simulink model "Dual_Three_Leg_Inverter_DPWMA"  (R2023b)
settings: Solver=ode45  StartTime=0.0  StopTime=0.5  RelTol=1e-3  EnableMultiTasking=on
libraries: spsSeriesRLCBranchLib x12, spsCurrentMeasurementLib x7, spsRMSLib x3, spsVoltageMeasurementLib x3, simulink x2, spsMeanLib x2, spsTHDLib x2, spsUniversalBridgeLib x2, spsDCVoltageSourceLib x1, spspowerguiLib x1
settings Model: SimulationMode=accelerator  Creator=Administrator  LastModifiedBy=Qu
settings SolverCC: AlgebraicLoopSolver=TrustRegion
settings DataIOCC: LimitDataPoints=on  SaveFormat=Array  SignalLoggingSaveFormat=ModelDataLogs  ReturnWorkspaceOutputs=off
settings OptimizationCC: ExpressionDepthLimit=2147483647  LifeSpan=inf
settings DebuggingCC: UnderspecifiedInitializationDetection=Classic  MergeDetectMultiDrivingBlocksExec=none  SolverPrmCheckMsg=warning  FcnCallInpInsideContextMsg=warning  UnconnectedInputMsg=warning  UnconnectedOutputMsg=warning  UnconnectedLineMsg=warning  StateNameClashWarn=warning  SFUnexpectedBacktrackingDiag=warning  SFNoUnconditionalDefaultTransitionDiag=warning  SFExecutionAtInitializationDiag=none  ArithmeticOperatorsInVariantConditions=warning
settings HardwareCC: ProdBitPerPointer=32  ProdBitPerSizeT=32  ProdBitPerPtrDiffT=32  ProdLargestAtomicFloat=None  ProdIntDivRoundTo=Undefined  ProdEndianess=Unspecified  ProdWordSize=32  ProdHWDeviceType=32-bit Generic
settings ModelReferenceCC: EnableRefExpFcnMdlSchedulingChecks=on  PropagateSignalLabelsOutOfModel=off
settings SFSimCC: SimUseLocalCustomCode=off  CustomCodeUndefinedFunction=UseInterfaceOnly
settings RTWCC: RTWUseLocalCustomCode=off
settings CodeAppCC: StateflowObjectComments=on
settings GRTTargetCC: TargetLangStandard=C89/C90 (ANSI)  CombineOutputUpdateFcns=off  GRTInterface=on
settings ConfigComp: CovMetricSettings=dw  CovSaveCumulativeToWorkspaceVar=on  CovSaveSingleToWorkspaceVar=on  CovExternalEMLEnable=off
settings SimscapeCC: SimscapeNormalizeSystem=off

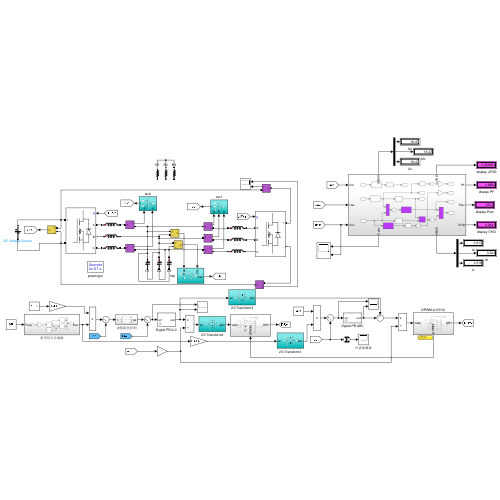
[thumbnail: Simulink's stored preview of the top-level diagram]
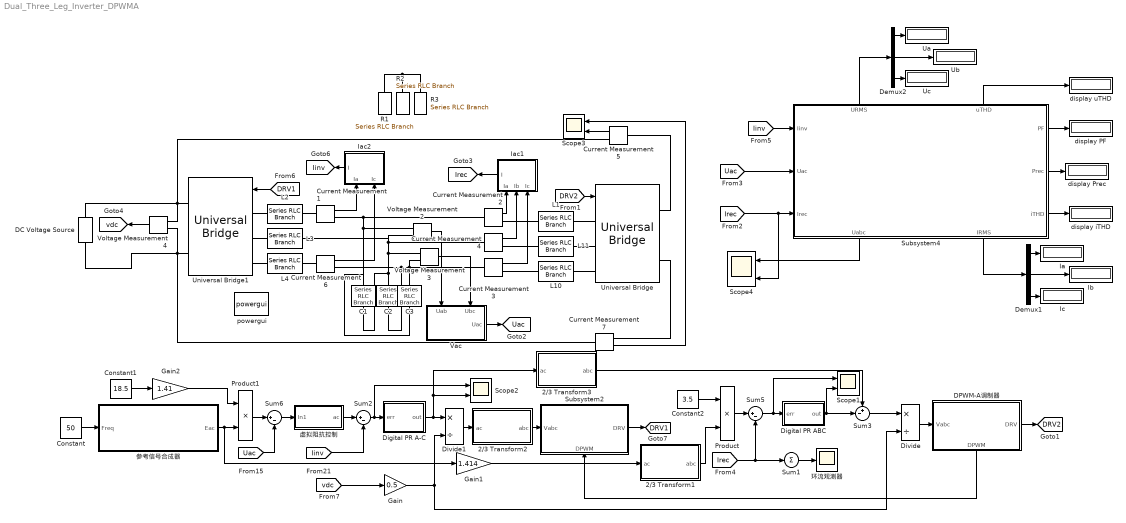
== system Dual_Three_Leg_Inverter_DPWMA ==
  2/3 Transform1 : Subsystem
      settings: PortSchema="{\"entries\":[{\"content\":{\"sides\":[{\"content\":{},\"type\":\"ConnectorPlacement.EquallySpacedRectSide\",\"uuid\":\"58c40194-9a95-4e39-952e-f878bde7484e\"},{\"content\":{\"side\":\"RIGHT\"},\"type\":\"ConnectorPlacement.EquallySpacedRectSide\",\"uuid\":\"f51692e8-3ff2-4d72-808d-3667196a4526\"},{\"content\":{\"connectorIds\":[\"In1\"],\"side\":\"TOP\"},\"type\":\"ConnectorPlacement.EquallySpacedRectSide\",\"uuid\":\"0aab136b-5da5-45c4-8998-999ebe8b7f2f\"},{\"content\":{\"connectorIds\":[\"Out1\"],\"side\":\"BOTTOM\"},\"type\":\"ConnectorPlacement.EquallySpacedRectSide\",\"uuid\":\"32f5f4a5-4ebb-496b-828d-b973bd46b44e\"}]},\"type\":\"ConnectorPlacement.EquallySpacedConnector\",\"uuid\":\"3ef81af7-d426-47fb-88e3-e33e58eebb83\"}],\"packageUris\":[\"http://schema.mathworks.com/mf0/Connector/R2020b\"],\"version\":\"1.0\"}"
  2/3 Transform2 : Subsystem
      settings: PortSchema="{\"entries\":[{\"content\":{\"sides\":[{\"content\":{},\"type\":\"ConnectorPlacement.EquallySpacedRectSide\",\"uuid\":\"58c40194-9a95-4e39-952e-f878bde7484e\"},{\"content\":{\"side\":\"RIGHT\"},\"type\":\"ConnectorPlacement.EquallySpacedRectSide\",\"uuid\":\"f51692e8-3ff2-4d72-808d-3667196a4526\"},{\"content\":{\"connectorIds\":[\"In1\"],\"side\":\"TOP\"},\"type\":\"ConnectorPlacement.EquallySpacedRectSide\",\"uuid\":\"0aab136b-5da5-45c4-8998-999ebe8b7f2f\"},{\"content\":{\"connectorIds\":[\"Out1\"],\"side\":\"BOTTOM\"},\"type\":\"ConnectorPlacement.EquallySpacedRectSide\",\"uuid\":\"32f5f4a5-4ebb-496b-828d-b973bd46b44e\"}]},\"type\":\"ConnectorPlacement.EquallySpacedConnector\",\"uuid\":\"3ef81af7-d426-47fb-88e3-e33e58eebb83\"}],\"packageUris\":[\"http://schema.mathworks.com/mf0/Connector/R2020b\"],\"version\":\"1.0\"}"
  2/3 Transform3 : Subsystem
      settings: PortSchema="{\"entries\":[{\"content\":{\"sides\":[{\"content\":{},\"type\":\"ConnectorPlacement.EquallySpacedRectSide\",\"uuid\":\"58c40194-9a95-4e39-952e-f878bde7484e\"},{\"content\":{\"side\":\"RIGHT\"},\"type\":\"ConnectorPlacement.EquallySpacedRectSide\",\"uuid\":\"f51692e8-3ff2-4d72-808d-3667196a4526\"},{\"content\":{\"connectorIds\":[\"In1\"],\"side\":\"TOP\"},\"type\":\"ConnectorPlacement.EquallySpacedRectSide\",\"uuid\":\"0aab136b-5da5-45c4-8998-999ebe8b7f2f\"},{\"content\":{\"connectorIds\":[\"Out1\"],\"side\":\"BOTTOM\"},\"type\":\"ConnectorPlacement.EquallySpacedRectSide\",\"uuid\":\"32f5f4a5-4ebb-496b-828d-b973bd46b44e\"}]},\"type\":\"ConnectorPlacement.EquallySpacedConnector\",\"uuid\":\"3ef81af7-d426-47fb-88e3-e33e58eebb83\"}],\"packageUris\":[\"http://schema.mathworks.com/mf0/Connector/R2020b\"],\"version\":\"1.0\"}"
  C1 : spsSeriesRLCBranchLib/Series RLC Branch  LConnTagsString=__new0  RConnTagsString=__new0  BranchType=C  Resistance=100  Inductance=1e-3  SetiL0=off  InitialCurrent=0  Capacitance=8e-6  Setx0=off  InitialVoltage=56  Measurements=None
  C2 : spsSeriesRLCBranchLib/Series RLC Branch  LConnTagsString=__new0  RConnTagsString=__new0  BranchType=C  Resistance=100  Inductance=1e-3  SetiL0=off  InitialCurrent=0  Capacitance=8e-6  Setx0=off  InitialVoltage=56  Measurements=None
  C3 : spsSeriesRLCBranchLib/Series RLC Branch  LConnTagsString=__new0  RConnTagsString=__new0  BranchType=C  Resistance=100  Inductance=1e-3  SetiL0=off  InitialCurrent=0  Capacitance=8e-6  Setx0=off  InitialVoltage=56  Measurements=None
  Constant : Constant  Value=50
  Constant1 : Constant  Value=18.5
  Constant2 : Constant  Value=3.5
  Current Measurement{1..7} (7 alike) : spsCurrentMeasurementLib/Current Measurement  PhasorSimulation=off  OutputType=Complex  PSBequivalent=0
  DC Voltage Source : spsDCVoltageSourceLib/DC Voltage Source  Amplitude=50  Measurements=None
  DPWM-A调制器 : Subsystem
      settings: PortSchema="{\"entries\":[{\"content\":{\"sides\":[{\"content\":{\"connectorIds\":[\"In1\"]},\"type\":\"ConnectorPlacement.EquallySpacedRectSide\",\"uuid\":\"1b921e88-89d9-40c8-80a6-19c9bba63005\"},{\"content\":{\"connectorIds\":[\"Out1\"],\"side\":\"RIGHT\"},\"type\":\"ConnectorPlacement.EquallySpacedRectSide\",\"uuid\":\"19f123f7-b197-44a6-b6a2-b5017f4a2a93\"},{\"content\":{\"side\":\"TOP\"},\"type\":\"ConnectorPlacement.EquallySpacedRectSide\",\"uuid\":\"1cf9155b-da68-48e1-b9a8-e44105d4bd88\"},{\"content\":{\"connectorIds\":[\"Out2\"],\"side\":\"BOTTOM\"},\"type\":\"ConnectorPlacement.EquallySpacedRectSide\",\"uuid\":\"2b44f05d-f684-4967-9c90-42e6d34a3f81\"}]},\"type\":\"ConnectorPlacement.EquallySpacedConnector\",\"uuid\":\"7b9a8e17-ffb5-4515-884d-b733a1796f36\"}],\"packageUris\":[\"http://schema.mathworks.com/mf0/Connector/R2020b\"],\"version\":\"1.0\"}"
  Demux1 : Demux  Outputs=3
  Demux2 : Demux  Outputs=3
  Digital PR A-C : Subsystem  mask{Kp=5, Kr=100, Wc=5, Ts=1/40000, Upper=80, Lower=-80}
      mask DialogControl ParameterGroupVar Prompt: 参数
  Digital PR ABC : Subsystem  mask{Kp=5, Kr=100, Wc=5, Ts=1/40000, Upper=80, Lower=-80}
      mask DialogControl ParameterGroupVar Prompt: 参数
  Divide : Product  Inputs=*/
  Divide1 : Product  Inputs=*/
  Gain : Gain  Gain=0.5
  Gain1 : Gain  Gain=1.414
  Gain2 : Gain  Gain=1.41
  Ia : Display
  Iac1 : Subsystem
      settings: PortSchema="{\"entries\":[{\"content\":{\"sides\":[{\"content\":{\"connectorIds\":[\"In1\",\"In2\",\"In3\"]},\"type\":\"ConnectorPlacement.EquallySpacedRectSide\",\"uuid\":\"58c40194-9a95-4e39-952e-f878bde7484e\"},{\"content\":{\"side\":\"RIGHT\"},\"type\":\"ConnectorPlacement.EquallySpacedRectSide\",\"uuid\":\"f51692e8-3ff2-4d72-808d-3667196a4526\"},{\"content\":{\"side\":\"TOP\"},\"type\":\"ConnectorPlacement.EquallySpacedRectSide\",\"uuid\":\"0aab136b-5da5-45c4-8998-999ebe8b7f2f\"},{\"content\":{\"connectorIds\":[\"Out1\"],\"side\":\"BOTTOM\"},\"type\":\"ConnectorPlacement.EquallySpacedRectSide\",\"uuid\":\"32f5f4a5-4ebb-496b-828d-b973bd46b44e\"}]},\"type\":\"ConnectorPlacement.EquallySpacedConnector\",\"uuid\":\"3ef81af7-d426-47fb-88e3-e33e58eebb83\"}],\"packageUris\":[\"http://schema.mathworks.com/mf0/Connector/R2020b\"],\"version\":\"1.0\"}"
  Iac2 : Subsystem
      settings: PortSchema="{\"entries\":[{\"content\":{\"sides\":[{\"content\":{\"connectorIds\":[\"In1\",\"In2\"]},\"type\":\"ConnectorPlacement.EquallySpacedRectSide\",\"uuid\":\"58c40194-9a95-4e39-952e-f878bde7484e\"},{\"content\":{\"side\":\"RIGHT\"},\"type\":\"ConnectorPlacement.EquallySpacedRectSide\",\"uuid\":\"f51692e8-3ff2-4d72-808d-3667196a4526\"},{\"content\":{\"side\":\"TOP\"},\"type\":\"ConnectorPlacement.EquallySpacedRectSide\",\"uuid\":\"0aab136b-5da5-45c4-8998-999ebe8b7f2f\"},{\"content\":{\"connectorIds\":[\"Out1\"],\"side\":\"BOTTOM\"},\"type\":\"ConnectorPlacement.EquallySpacedRectSide\",\"uuid\":\"32f5f4a5-4ebb-496b-828d-b973bd46b44e\"}]},\"type\":\"ConnectorPlacement.EquallySpacedConnector\",\"uuid\":\"3ef81af7-d426-47fb-88e3-e33e58eebb83\"}],\"packageUris\":[\"http://schema.mathworks.com/mf0/Connector/R2020b\"],\"version\":\"1.0\"}"
  Ib : Display
  Ic : Display
  L1 : spsSeriesRLCBranchLib/Series RLC Branch  LConnTagsString=__new0  RConnTagsString=__new0  BranchType=L  Resistance=1  Inductance=3e-4  SetiL0=off  InitialCurrent=0  Capacitance=2e-3  Setx0=off  InitialVoltage=0  Measurements=None
  L10 : spsSeriesRLCBranchLib/Series RLC Branch  LConnTagsString=__new0  RConnTagsString=__new0  BranchType=L  Resistance=1  Inductance=3e-4  SetiL0=off  InitialCurrent=0  Capacitance=2e-3  Setx0=off  InitialVoltage=0  Measurements=None
  L11 : spsSeriesRLCBranchLib/Series RLC Branch  LConnTagsString=__new0  RConnTagsString=__new0  BranchType=L  Resistance=1  Inductance=3e-4  SetiL0=off  InitialCurrent=0  Capacitance=2e-3  Setx0=off  InitialVoltage=0  Measurements=None
  L2 : spsSeriesRLCBranchLib/Series RLC Branch  LConnTagsString=__new0  RConnTagsString=__new0  BranchType=L  Resistance=0.1  Inductance=3e-4  SetiL0=off  InitialCurrent=0  Capacitance=2e-3  Setx0=off  InitialVoltage=0  Measurements=None
  L3 : spsSeriesRLCBranchLib/Series RLC Branch  LConnTagsString=__new0  RConnTagsString=__new0  BranchType=L  Resistance=0.1  Inductance=3e-4  SetiL0=off  InitialCurrent=0  Capacitance=2e-3  Setx0=off  InitialVoltage=0  Measurements=None
  L4 : spsSeriesRLCBranchLib/Series RLC Branch  LConnTagsString=__new0  RConnTagsString=__new0  BranchType=L  Resistance=0.1  Inductance=3e-4  SetiL0=off  InitialCurrent=0  Capacitance=2e-3  Setx0=off  InitialVoltage=0  Measurements=None
  Product : Product
  Product1 : Product
  R1 : spsSeriesRLCBranchLib/Series RLC Branch  LConnTagsString=__new0  RConnTagsString=__new0  BranchType=R  Resistance=10  Inductance=1e-3  SetiL0=off  InitialCurrent=0  Capacitance=2e-3  Setx0=on  InitialVoltage=540  Measurements=None
  R2 : spsSeriesRLCBranchLib/Series RLC Branch  LConnTagsString=__new0  RConnTagsString=__new0  BranchType=R  Resistance=10  Inductance=1e-3  SetiL0=off  InitialCurrent=0  Capacitance=2e-3  Setx0=on  InitialVoltage=540  Measurements=None
  R3 : spsSeriesRLCBranchLib/Series RLC Branch  LConnTagsString=__new0  RConnTagsString=__new0  BranchType=R  Resistance=10  Inductance=1e-3  SetiL0=off  InitialCurrent=0  Capacitance=2e-3  Setx0=on  InitialVoltage=540  Measurements=None
  Scope{1..4} (4 alike) : Scope  NumInputPorts=2
  Subsystem2 : Subsystem
      settings: PortSchema="{\"entries\":[{\"content\":{\"sides\":[{\"content\":{\"connectorIds\":[\"In1\"]},\"type\":\"ConnectorPlacement.EquallySpacedRectSide\",\"uuid\":\"de8b90f0-7b55-4abd-a179-300fa705da97\"},{\"content\":{\"connectorIds\":[\"Out1\"],\"side\":\"RIGHT\"},\"type\":\"ConnectorPlacement.EquallySpacedRectSide\",\"uuid\":\"0792874a-d250-4054-8a74-d5389a9b2639\"},{\"content\":{\"side\":\"TOP\"},\"type\":\"ConnectorPlacement.EquallySpacedRectSide\",\"uuid\":\"613a9447-7ac5-4140-b452-30bec5459d5a\"},{\"content\":{\"connectorIds\":[\"In2\"],\"side\":\"BOTTOM\"},\"type\":\"ConnectorPlacement.EquallySpacedRectSide\",\"uuid\":\"fd3fd695-8830-4e72-9238-e853f444166a\"}]},\"type\":\"ConnectorPlacement.EquallySpacedConnector\",\"uuid\":\"d7512945-9f99-49d8-b46f-637000ed2988\"}],\"packageUris\":[\"http://schema.mathworks.com/mf0/Connector/R2020b\"],\"version\":\"1.0\"}"
  Subsystem4 : Subsystem
      settings: PortSchema="{\"entries\":[{\"content\":{\"sides\":[{\"content\":{\"connectorIds\":[\"In1\",\"In2\",\"In3\"]},\"type\":\"ConnectorPlacement.EquallySpacedRectSide\",\"uuid\":\"8f3b7bf1-7c44-4492-a357-aa6e3e6d66a4\"},{\"content\":{\"connectorIds\":[\"Out1\",\"Out2\",\"Out3\"],\"side\":\"RIGHT\"},\"type\":\"ConnectorPlacement.EquallySpacedRectSide\",\"uuid\":\"7ae784cf-6bcf-4684-9c07-1770fc60c8a0\"},{\"content\":{\"connectorIds\":[\"Out6\",\"Out7\"],\"side\":\"TOP\"},\"type\":\"ConnectorPlacement.EquallySpacedRectSide\",\"uuid\":\"0e016931-6232-4ad6-afe9-572a0571336f\"},{\"content\":{\"connectorIds\":[\"Out4\",\"Out5\"],\"side\":\"BOTTOM\"},\"type\":\"ConnectorPlacement.EquallySpacedRectSide\",\"uuid\":\"ef67c6ee-ba81-4705-af34-81581e7e9907\"}]},\"type\":\"ConnectorPlacement.EquallySpacedConnector\",\"uuid\":\"922af512-c0ff-443f-816c-194775a78dc8\"}],\"packageUris\":[\"http://schema.mathworks.com/mf0/Connector/R2020b\"],\"version\":\"1.0\"}"
  Sum1 : Sum  Inputs=+
  Sum2 : Sum  Inputs=|+-
  Sum3 : Sum  Inputs=+-|
  Sum5 : Sum  Inputs=|+-
  Sum6 : Sum  Inputs=|+-
  Ua : Display
  Ub : Display
  Uc : Display
  Universal Bridge : spsUniversalBridgeLib/Universal Bridge  Arms=3  SnubberResistance=1e5  SnubberCapacitance=inf  Device=MOSFET / Diodes  Ron=1e-3  Lon=0  ForwardVoltages="[  0  0  ]"  ForwardVoltage=0  GTOparameters=[ 10e-6 , 20e-6 ]  IGBTparameters=[ 1e-6 , 2e-6 ]  Measurements=None  Measurements_2=None  converterType=Rectifier
  Universal Bridge1 : spsUniversalBridgeLib/Universal Bridge  Arms=3  SnubberResistance=1e5  SnubberCapacitance=inf  Device=MOSFET / Diodes  Ron=1e-3  Lon=0  ForwardVoltages="[  0  0  ]"  ForwardVoltage=0  GTOparameters=[ 10e-6 , 20e-6 ]  IGBTparameters=[ 1e-6 , 2e-6 ]  Measurements=None  Measurements_2=None  converterType=Rectifier
  Vac : Subsystem
      settings: PortSchema="{\"entries\":[{\"content\":{\"sides\":[{\"content\":{\"connectorIds\":[\"In1\",\"In2\"]},\"type\":\"ConnectorPlacement.EquallySpacedRectSide\",\"uuid\":\"58c40194-9a95-4e39-952e-f878bde7484e\"},{\"content\":{\"connectorIds\":[],\"side\":\"RIGHT\"},\"type\":\"ConnectorPlacement.EquallySpacedRectSide\",\"uuid\":\"f51692e8-3ff2-4d72-808d-3667196a4526\"},{\"content\":{\"connectorIds\":[],\"side\":\"TOP\"},\"type\":\"ConnectorPlacement.EquallySpacedRectSide\",\"uuid\":\"0aab136b-5da5-45c4-8998-999ebe8b7f2f\"},{\"content\":{\"connectorIds\":[\"Out1\"],\"side\":\"BOTTOM\"},\"type\":\"ConnectorPlacement.EquallySpacedRectSide\",\"uuid\":\"185ce796-68e2-4136-8080-97dc86d2ba54\"}]},\"type\":\"ConnectorPlacement.EquallySpacedConnector\",\"uuid\":\"3ef81af7-d426-47fb-88e3-e33e58eebb83\"}],\"packageUris\":[\"http://schema.mathworks.com/mf0/Connector/R2020b\"],\"version\":\"1.0\"}"
  Voltage Measurement2 : spsVoltageMeasurementLib/Voltage Measurement  PhasorSimulation=off  OutputType=Complex  PSBequivalent=0
  Voltage Measurement3 : spsVoltageMeasurementLib/Voltage Measurement  PhasorSimulation=off  OutputType=Complex  PSBequivalent=0
  Voltage Measurement4 : spsVoltageMeasurementLib/Voltage Measurement  PhasorSimulation=off  OutputType=Complex  PSBequivalent=0
  display PF : Display
  display Prec : Display
  display iTHD : Display
  display uTHD : Display
  powergui : spspowerguiLib/powergui  Priority=1  SimulationMode=Discrete  SampleTime=2e-7  frequency=60  Iterations=50  frequencyindice=0  Pbase=100e6  ErrMax=1e-4  UnitsV=kV  UnitsW=MW  buscounter=0  FunctionMessages=off  echomessages=off  EnableUseOfTLC=off  CurrentSourceSwitches=off  DisableSnubberDevices=off  DisableRonSwitches=off  DisableVfSwitches=off  DisplayEquations=off  AutomaticDiscreteSolvers=off  SolverType=Tustin  Interpol=off  ExternalGateDelay=off  methode=off  Ts=0  x0status=blocks  SPID=off  SwTol=0  HookPort=off  NonlinearTolerance=1e-4  nMaxIteration=100  ContinueOnMaxIteration=off  RestoreLinks=warning  ResistiveCurrentMeasurement=off  Frange=[0:2:500]  Ylog=off  Xlog=on  ShowGrid=off  save=off  variable=ZData  structure=0  ZoomFFT=off  StartTime=0.0  cycles=1  DisplayStyle=1  fundamental=60  FreqAxis=off  MaxFrequency=1000  frequencyindicesteady=1  RmsSteady=1  display=off
  参考信号合成器 : Subsystem
  环流观测器 : Scope
  虚拟阻抗控制 : Subsystem
  tag scope: DRV1=global, DRV2=global, Iinv=global, Irec=global, Uac=global, vdc=global
  wires:
  [DRV2] -> Universal Bridge/1
  [Irec] -> Sum1/1, Sum5/2
  Sum5/1 -> Scope1/1, Digital PR ABC/1(err)
  Digital PR ABC/1(out) -> Scope1/2, Sum3/2
  Voltage Measurement2/1 -> Vac/1(Uab)
  Voltage Measurement3/1 -> Vac/2(Ubc)
  Vac/1(Uac) -> [Uac]
  Subsystem4/1(PF) -> display PF/1
  Subsystem4/3(iTHD) -> display iTHD/1
  [Iinv] -> Subsystem4/1(Iinv)
  Product/1 -> Sum5/1
  Sum3/1 -> Divide/1
  [Irec] -> Scope4/2, Subsystem4/3(Irec)
  [Uac] -> Subsystem4/2(Uac)
  Current Measurement1/1 -> Iac2/2(Ia)
  Iac2/1(I) -> [Iinv]
  Constant/1 -> 参考信号合成器/1(Freq)
  Sum6/1 -> 虚拟阻抗控制/1(In1)
  [Iinv] -> Sum2/2
  [Uac] -> Sum6/2
  参考信号合成器/1(Eac) -> Gain1/1, Product1/2
  Gain2/1 -> Product1/1
  Constant1/1 -> Gain2/1
  Product1/1 -> Sum6/1
  [DRV1] -> Universal Bridge1/1
  Current Measurement2/1 -> Iac1/3(Ia)
  Iac1/1(I) -> [Irec]
  Current Measurement3/1 -> Iac1/1(Ic)
  Current Measurement4/1 -> Iac1/2(Ib)
  Subsystem2/1(DRV) -> [DRV1]
  Voltage Measurement4/1 -> [vdc]
  Current Measurement5/1 -> Scope3/2
  Current Measurement7/1 -> Scope3/1
  Constant2/1 -> Product/1
  Current Measurement6/1 -> Iac2/1(Ic)
  Sum2/1 -> Scope2/1, Digital PR A-C/1(err)
  2/3 Transform1/1(abc) -> Product/2
  虚拟阻抗控制/1(ac) -> Sum2/1
  Divide1/1 -> 2/3 Transform2/1(ac)
  DPWM-A调制器/1(DRV) -> [DRV2]
  [vdc] -> Gain/1
  Gain/1 -> Divide/2, Divide1/2
  Divide/1 -> DPWM-A调制器/1(Vabc)
  Sum1/1 -> 环流观测器/1
  2/3 Transform2/1(abc) -> Subsystem2/1(Vabc)
  2/3 Transform3/1(abc) -> Sum3/1
  Digital PR A-C/1(out) -> Divide1/1, 2/3 Transform3/1(ac), Scope2/2
  Demux2/3 -> Uc/1
  Demux2/1 -> Ua/1
  Demux2/2 -> Ub/1
  Subsystem4/6(URMS) -> Demux2/1
  Subsystem4/2(Prec) -> display Prec/1
  Subsystem4/7(uTHD) -> display uTHD/1
  Subsystem4/4(Uabc) -> Scope4/1
  Subsystem4/5(IRMS) -> Demux1/1
  Demux1/2 -> Ib/1
  Demux1/1 -> Ia/1
  Demux1/3 -> Ic/1
  Gain1/1 -> 2/3 Transform1/1(ac)
  DPWM-A调制器/2(DPWM) -> Subsystem2/2(DPWM)
  connections:
  L1/RConn1 -- Universal Bridge/LConn1
  L11/RConn1 -- Universal Bridge/LConn2
  L2/RConn1 -- Current Measurement1/LConn1
  Current Measurement1/RConn1 -- Current Measurement2/LConn1 -- C3/RConn1 -- C1/LConn1 -- Voltage Measurement2/LConn1
  Current Measurement2/RConn1 -- L1/LConn1
  L10/RConn1 -- Universal Bridge/LConn3
  Universal Bridge1/LConn1 -- L2/LConn1
  L3/LConn1 -- Universal Bridge1/LConn2
  L4/LConn1 -- Universal Bridge1/LConn3
  L4/RConn1 -- Current Measurement6/LConn1
  C2/LConn1 -- Current Measurement4/LConn1 -- Voltage Measurement2/LConn2 -- L3/RConn1 -- Voltage Measurement3/LConn1 -- C1/RConn1
  C3/LConn1 -- Current Measurement3/LConn1 -- Voltage Measurement3/LConn2 -- Current Measurement6/RConn1 -- C2/RConn1
  Current Measurement3/RConn1 -- L10/LConn1
  Current Measurement4/RConn1 -- L11/LConn1
  Voltage Measurement4/LConn1 -- Universal Bridge1/RConn1 -- Current Measurement5/RConn1 -- DC Voltage Source/RConn1
  Voltage Measurement4/LConn2 -- Current Measurement7/LConn1 -- DC Voltage Source/LConn1 -- Universal Bridge1/RConn2
  Current Measurement5/LConn1 -- Universal Bridge/RConn1
  Current Measurement7/RConn1 -- Universal Bridge/RConn2
  R1/RConn1 -- R3/RConn1 -- R2/RConn1

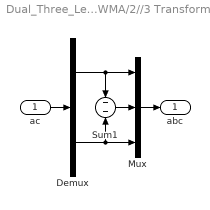
== system Dual_Three_Leg_Inverter_DPWMA/2//3 Transform1 ==
  ac : Inport
  Demux : Demux  Outputs=2
  Mux : Mux  Inputs=3
  Sum1 : Sum  Inputs=-|-
  abc : Outport
  wires:
  Demux/2 -> Mux/3, Sum1/2
  ac/1 -> Demux/1
  Demux/1 -> Mux/1, Sum1/1
  Mux/1 -> abc/1
  Sum1/1 -> Mux/2

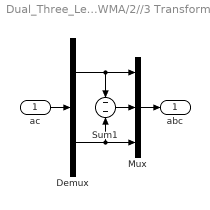
== system Dual_Three_Leg_Inverter_DPWMA/2//3 Transform2 ==
  ac : Inport
  Demux : Demux  Outputs=2
  Mux : Mux  Inputs=3
  Sum1 : Sum  Inputs=-|-
  abc : Outport
  wires:
  Sum1/1 -> Mux/2
  Mux/1 -> abc/1
  Demux/1 -> Sum1/1, Mux/1
  ac/1 -> Demux/1
  Demux/2 -> Sum1/2, Mux/3

== system Dual_Three_Leg_Inverter_DPWMA/2//3 Transform3 ==
  ac : Inport
  Demux : Demux  Outputs=2
  Mux : Mux  Inputs=3
  Sum1 : Sum  Inputs=-|-
  abc : Outport
  wires:
  Sum1/1 -> Mux/2
  Mux/1 -> abc/1
  Demux/1 -> Sum1/1, Mux/1
  ac/1 -> Demux/1
  Demux/2 -> Sum1/2, Mux/3

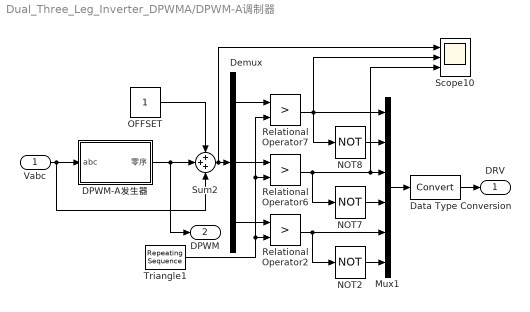
== system Dual_Three_Leg_Inverter_DPWMA/DPWM-A调制器 ==
  Vabc : Inport
  DPWM-A发生器 : Subsystem
  Data Type Conversion : DataTypeConversion  SaturateOnIntegerOverflow=off  RndMeth=Floor
  Demux : Demux  Outputs=3
  Mux1 : Mux  Inputs=6
  NOT2 : Logic  Operator=NOT  IconShape=distinctive  AllPortsSameDT=off  OutDataTypeStr=boolean
  NOT7 : Logic  Operator=NOT  IconShape=distinctive  AllPortsSameDT=off  OutDataTypeStr=boolean
  NOT8 : Logic  Operator=NOT  IconShape=distinctive  AllPortsSameDT=off  OutDataTypeStr=boolean
  OFFSET : Constant
  Relational Operator2 : RelationalOperator  Operator=>  OutDataTypeStr=boolean  InputSameDT=off
  Relational Operator6 : RelationalOperator  Operator=>  OutDataTypeStr=boolean  InputSameDT=off
  Relational Operator7 : RelationalOperator  Operator=>  OutDataTypeStr=boolean  InputSameDT=off
  Scope10 : Scope  NumInputPorts=3
  Sum2 : Sum  Inputs=+++
  Triangle1 : simulink/Sources/Repeating Sequence  rep_seq_t=[0 1/20000/2 1/20000]  rep_seq_y=[0 2 0]
  DRV : Outport
  DPWM : Outport  Port=2
  wires:
  Vabc/1 -> DPWM-A发生器/1(abc), Sum2/3
  Relational Operator6/1 -> Scope10/3, Mux1/3, NOT7/1
  NOT7/1 -> Mux1/4
  Relational Operator7/1 -> NOT8/1, Scope10/2, Mux1/1
  Triangle1/1 -> Relational Operator2/2, Relational Operator7/2, Relational Operator6/2
  NOT8/1 -> Mux1/2
  Relational Operator2/1 -> Mux1/5, NOT2/1
  NOT2/1 -> Mux1/6
  Demux/1 -> Relational Operator7/1
  Demux/2 -> Relational Operator6/1
  Demux/3 -> Relational Operator2/1
  Sum2/1 -> Scope10/1, Demux/1
  Mux1/1 -> Data Type Conversion/1
  Data Type Conversion/1 -> DRV/1
  OFFSET/1 -> Sum2/1
  DPWM-A发生器/1(零序) -> DPWM/1, Sum2/2

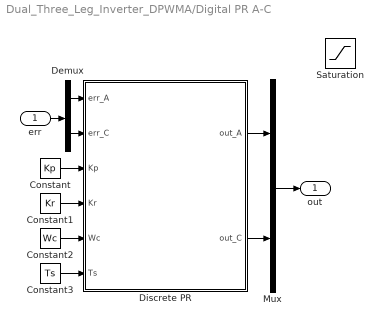
== system Dual_Three_Leg_Inverter_DPWMA/Digital PR A-C ==
  err : Inport
  Constant : Constant  Value=Kp
  Constant1 : Constant  Value=Kr
  Constant2 : Constant  Value=Wc
  Constant3 : Constant  Value=Ts
  Demux : Demux  Outputs=2
  Discrete PR : MATLAB Function  TreatAsAtomicUnit=on
  Mux : Mux  Inputs=2
  Saturation : Saturate  UpperLimit=Upper  LowerLimit=Lower
  out : Outport
  wires:
  Constant1/1 -> Discrete PR/4(Kr)
  Constant3/1 -> Discrete PR/6(Ts)
  Constant/1 -> Discrete PR/3(Kp)
  Constant2/1 -> Discrete PR/5(Wc)
  Demux/1 -> Discrete PR/1(err_A)
  err/1 -> Demux/1
  Demux/2 -> Discrete PR/2(err_C)
  Discrete PR/1(out_A) -> Mux/1
  Discrete PR/2(out_C) -> Mux/2
  Mux/1 -> out/1

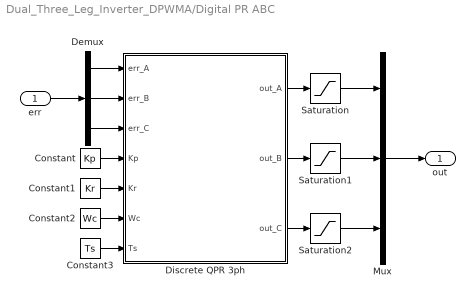
== system Dual_Three_Leg_Inverter_DPWMA/Digital PR ABC ==
  err : Inport
  Constant : Constant  Value=Kp
  Constant1 : Constant  Value=Kr
  Constant2 : Constant  Value=Wc
  Constant3 : Constant  Value=Ts
  Demux : Demux  Outputs=3
  Discrete QPR 3ph : MATLAB Function  TreatAsAtomicUnit=on
  Mux : Mux  Inputs=3
  Saturation : Saturate  UpperLimit=Upper  LowerLimit=Lower
  Saturation1 : Saturate  UpperLimit=Upper  LowerLimit=Lower
  Saturation2 : Saturate  UpperLimit=Upper  LowerLimit=Lower
  out : Outport
  wires:
  Discrete QPR 3ph/1(out_A) -> Saturation/1
  Constant1/1 -> Discrete QPR 3ph/5(Kr)
  Constant3/1 -> Discrete QPR 3ph/7(Ts)
  Constant/1 -> Discrete QPR 3ph/4(Kp)
  Constant2/1 -> Discrete QPR 3ph/6(Wc)
  Discrete QPR 3ph/2(out_B) -> Saturation1/1
  Discrete QPR 3ph/3(out_C) -> Saturation2/1
  Demux/2 -> Discrete QPR 3ph/2(err_B)
  Demux/3 -> Discrete QPR 3ph/3(err_C)
  Demux/1 -> Discrete QPR 3ph/1(err_A)
  err/1 -> Demux/1
  Saturation2/1 -> Mux/3
  Saturation1/1 -> Mux/2
  Saturation/1 -> Mux/1
  Mux/1 -> out/1

== system Dual_Three_Leg_Inverter_DPWMA/Iac1 ==
  Ic : Inport
  Ib : Inport  Port=2
  Ia : Inport  Port=3
  Mux : Mux  Inputs=3
  I : Outport
  wires:
  Ia/1 -> Mux/1
  Ib/1 -> Mux/2
  Mux/1 -> I/1
  Ic/1 -> Mux/3

== system Dual_Three_Leg_Inverter_DPWMA/Iac2 ==
  Ic : Inport
  Ia : Inport  Port=2
  Mux : Mux  Inputs=2
  I : Outport
  wires:
  Mux/1 -> I/1
  Ia/1 -> Mux/1
  Ic/1 -> Mux/2

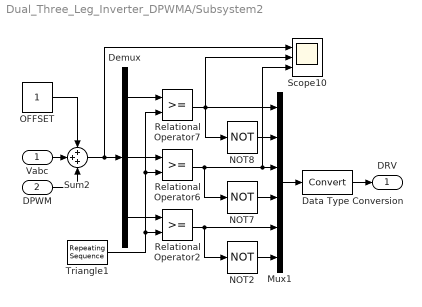
== system Dual_Three_Leg_Inverter_DPWMA/Subsystem2 ==
  Vabc : Inport
  DPWM : Inport  Port=2
  Data Type Conversion : DataTypeConversion  SaturateOnIntegerOverflow=off  RndMeth=Floor
  Demux : Demux  Outputs=3
  Mux1 : Mux  Inputs=6
  NOT2 : Logic  Operator=NOT  IconShape=distinctive  AllPortsSameDT=off  OutDataTypeStr=boolean
  NOT7 : Logic  Operator=NOT  IconShape=distinctive  AllPortsSameDT=off  OutDataTypeStr=boolean
  NOT8 : Logic  Operator=NOT  IconShape=distinctive  AllPortsSameDT=off  OutDataTypeStr=boolean
  OFFSET : Constant
  Relational Operator2 : RelationalOperator  OutDataTypeStr=boolean  InputSameDT=off
  Relational Operator6 : RelationalOperator  OutDataTypeStr=boolean  InputSameDT=off
  Relational Operator7 : RelationalOperator  OutDataTypeStr=boolean  InputSameDT=off
  Scope10 : Scope  NumInputPorts=3
  Sum2 : Sum  Inputs=+++
  Triangle1 : simulink/Sources/Repeating Sequence  rep_seq_t=[0 1/20000/2 1/20000]  rep_seq_y=[0 2 0]
  DRV : Outport
  wires:
  OFFSET/1 -> Sum2/1
  Data Type Conversion/1 -> DRV/1
  Mux1/1 -> Data Type Conversion/1
  Sum2/1 -> Scope10/1, Demux/1
  Demux/3 -> Relational Operator2/1
  Demux/2 -> Relational Operator6/1
  Demux/1 -> Relational Operator7/1
  NOT2/1 -> Mux1/6
  Relational Operator2/1 -> NOT2/1, Mux1/5
  NOT8/1 -> Mux1/2
  Relational Operator7/1 -> NOT8/1, Scope10/2, Mux1/1
  NOT7/1 -> Mux1/4
  Relational Operator6/1 -> NOT7/1, Scope10/3, Mux1/3
  DPWM/1 -> Sum2/3
  Vabc/1 -> Sum2/2
  Triangle1/1 -> Relational Operator7/2, Relational Operator6/2, Relational Operator2/2

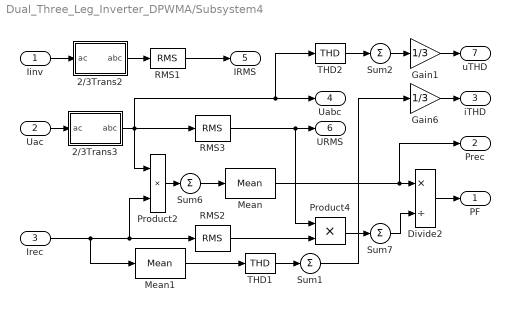
== system Dual_Three_Leg_Inverter_DPWMA/Subsystem4 ==
  Iinv : Inport
  Uac : Inport  Port=2
  Irec : Inport  Port=3
  2/3Trans2 : Subsystem
  2/3Trans3 : Subsystem
  Divide2 : Product  Inputs=*/
  Gain1 : Gain  Gain=1/3
  Gain6 : Gain  Gain=1/3
  Mean : spsMeanLib/Mean  Freq=100  Vinit=0  Ts=0
  Mean1 : spsMeanLib/Mean  Freq=5000  Vinit=0  Ts=0
  Product2 : Product
  Product4 : Product
  RMS1 : spsRMSLib/RMS  TrueRMS=on  Freq=50  RMSInit=0  Ts=0
  RMS2 : spsRMSLib/RMS  TrueRMS=on  Freq=50  RMSInit=0  Ts=0
  RMS3 : spsRMSLib/RMS  TrueRMS=on  Freq=50  RMSInit=0  Ts=0
  Sum{1..2,6..7} (4 alike) : Sum  Inputs=+
  THD1 : spsTHDLib/THD  Freq=50  Ts=0
  THD2 : spsTHDLib/THD  Freq=50  Ts=0
  PF : Outport
  Prec : Outport  Port=2
  iTHD : Outport  Port=3
  Uabc : Outport  Port=4
  IRMS : Outport  Port=5
  URMS : Outport  Port=6
  uTHD : Outport  Port=7
  wires:
  RMS1/1 -> IRMS/1
  2/3Trans2/1(abc) -> RMS1/1
  Iinv/1 -> 2/3Trans2/1(ac)
  Irec/1 -> Mean1/1, Product2/2, RMS2/1
  Product2/1 -> Sum6/1
  2/3Trans3/1(abc) -> Uabc/1, THD2/1, Product2/1, RMS3/1
  Uac/1 -> 2/3Trans3/1(ac)
  Product4/1 -> Sum7/1
  Sum7/1 -> Divide2/2
  RMS3/1 -> URMS/1, Product4/1
  THD1/1 -> Sum1/1
  RMS2/1 -> Product4/2
  Divide2/1 -> PF/1
  Sum6/1 -> Mean/1
  Gain6/1 -> iTHD/1
  Mean/1 -> Prec/1, Divide2/1
  Sum1/1 -> Gain6/1
  THD2/1 -> Sum2/1
  Sum2/1 -> Gain1/1
  Gain1/1 -> uTHD/1
  Mean1/1 -> THD1/1

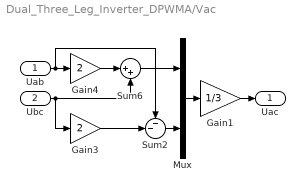
== system Dual_Three_Leg_Inverter_DPWMA/Vac ==
  Uab : Inport
  Ubc : Inport  Port=2
  Gain1 : Gain  Gain=1/3
  Gain3 : Gain  Gain=2
  Gain4 : Gain  Gain=2
  Mux : Mux  Inputs=2
  Sum2 : Sum  Inputs=--|
  Sum6 : Sum  Inputs=|++
  Uac : Outport
  wires:
  Uab/1 -> Sum2/1, Gain4/1
  Gain4/1 -> Sum6/1
  Ubc/1 -> Gain3/1, Sum6/2
  Gain3/1 -> Sum2/2
  Mux/1 -> Gain1/1
  Gain1/1 -> Uac/1
  Sum6/1 -> Mux/1
  Sum2/1 -> Mux/2

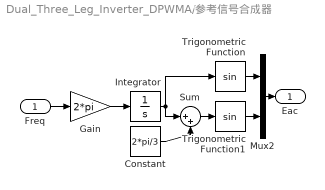
== system Dual_Three_Leg_Inverter_DPWMA/参考信号合成器 ==
  Freq : Inport
  Constant : Constant  Value=2*pi/3
  Gain : Gain  Gain=2*pi
  Integrator : Integrator  WrapState=on  WrappedStateUpperValue=2*pi  WrappedStateLowerValue=0
  Mux2 : Mux  Inputs=2
  Sum : Sum  Inputs=|++
  Trigonometric Function : Trigonometry
  Trigonometric Function1 : Trigonometry
  Eac : Outport
  wires:
  Gain/1 -> Integrator/1
  Freq/1 -> Gain/1
  Integrator/1 -> Trigonometric Function/1, Sum/1
  Constant/1 -> Sum/2
  Sum/1 -> Trigonometric Function1/1
  Trigonometric Function/1 -> Mux2/1
  Mux2/1 -> Eac/1
  Trigonometric Function1/1 -> Mux2/2

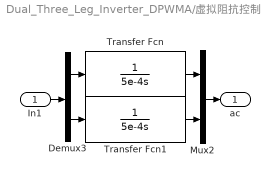
== system Dual_Three_Leg_Inverter_DPWMA/虚拟阻抗控制 ==
  In1 : Inport
  Demux3 : Demux  Outputs=2
  Mux2 : Mux  Inputs=2
  Transfer Fcn : TransferFcn  Denominator=[5e-4 0]
  Transfer Fcn1 : TransferFcn  Denominator=[5e-4 0]
  ac : Outport
  wires:
  Transfer Fcn/1 -> Mux2/1
  Mux2/1 -> ac/1
  Demux3/1 -> Transfer Fcn/1
  In1/1 -> Demux3/1
  Demux3/2 -> Transfer Fcn1/1
  Transfer Fcn1/1 -> Mux2/2

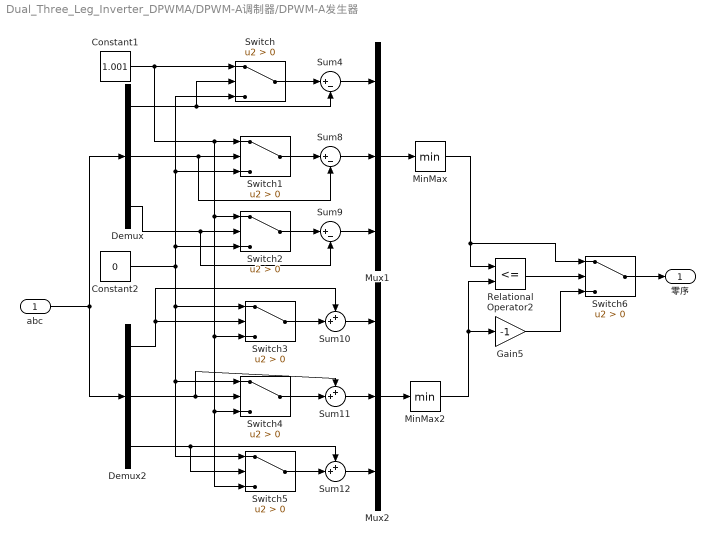
== system Dual_Three_Leg_Inverter_DPWMA/DPWM-A调制器/DPWM-A发生器 ==
  abc : Inport
  Constant1 : Constant  Value=1.001
  Constant2 : Constant  Value=0
  Demux : Demux  Outputs=3
  Demux2 : Demux  Outputs=3
  Gain5 : Gain  Gain=-1
  MinMax : MinMax
  MinMax2 : MinMax
  Mux1 : Mux  Inputs=3
  Mux2 : Mux  Inputs=3
  Relational Operator2 : RelationalOperator  Operator=<=  OutDataTypeStr=boolean  InputSameDT=off
  Sum10 : Sum  Inputs=++|
  Sum11 : Sum  Inputs=++|
  Sum12 : Sum  Inputs=++|
  Sum4 : Sum  Inputs=|+-
  Sum8 : Sum  Inputs=|+-
  Sum9 : Sum  Inputs=|+-
  Switch{,1..6} (7 alike) : Switch  Criteria=u2 > Threshold  SaturateOnIntegerOverflow=off  InputSameDT=off
  零序 : Outport
  wires:
  Switch1/1 -> Sum8/1
  Constant1/1 -> Switch5/3, Switch4/3, Switch3/3, Switch2/1, Switch1/1, Switch/1
  Constant2/1 -> Switch1/3, Switch/3, Switch2/3, Switch5/1, Switch4/1, Switch3/1
  Demux2/2 -> Sum11/1, Switch4/2
  Sum9/1 -> Mux1/3
  Switch2/1 -> Sum9/1
  MinMax/1 -> Switch6/1, Relational Operator2/1
  Relational Operator2/1 -> Switch6/2
  Mux1/1 -> MinMax/1
  Mux2/1 -> MinMax2/1
  Sum10/1 -> Mux2/1
  Sum11/1 -> Mux2/2
  Switch/1 -> Sum4/1
  Demux/1 -> Sum4/2, Switch/2
  Demux2/1 -> Sum10/1, Switch3/2
  Demux/3 -> Sum9/2, Switch2/2
  Sum12/1 -> Mux2/3
  Gain5/1 -> Switch6/3
  Switch4/1 -> Sum11/2
  Demux/2 -> Sum8/2, Switch1/2
  MinMax2/1 -> Gain5/1, Relational Operator2/2
  Switch5/1 -> Sum12/2
  Demux2/3 -> Switch5/2, Sum12/1
  Sum8/1 -> Mux1/2
  Sum4/1 -> Mux1/1
  Switch3/1 -> Sum10/2
  abc/1 -> Demux/1, Demux2/1
  Switch6/1 -> 零序/1

== system Dual_Three_Leg_Inverter_DPWMA/Subsystem4/2//3Trans2 ==
  ac : Inport
  Demux2 : Demux  Outputs=2
  Mux1 : Mux  Inputs=3
  Sum2 : Sum  Inputs=-|-
  abc : Outport
  wires:
  Sum2/1 -> Mux1/2
  Demux2/1 -> Sum2/1, Mux1/1
  Demux2/2 -> Sum2/2, Mux1/3
  Mux1/1 -> abc/1
  ac/1 -> Demux2/1

== system Dual_Three_Leg_Inverter_DPWMA/Subsystem4/2//3Trans3 ==
  ac : Inport
  Demux2 : Demux  Outputs=2
  Mux1 : Mux  Inputs=3
  Sum2 : Sum  Inputs=-|-
  abc : Outport
  wires:
  ac/1 -> Demux2/1
  Mux1/1 -> abc/1
  Demux2/2 -> Mux1/3, Sum2/2
  Demux2/1 -> Mux1/1, Sum2/1
  Sum2/1 -> Mux1/2

== matlab function Dual_Three_Leg_Inverter_DPWMA/Digital PR A-C/Discrete PR ==
  settings: updateMethod=DISCRETE  sampleTime=Ts
  data: err_A input; err_C input; out_A output; Kp input; Kr input; Wc input; Ts input; out_C output
function [out_A, out_C] = fcn(err_A, err_C, Kp, Kr, Wc, Ts)

W0 = 50*2*pi;

%%定义三相静态变量
persistent err_A1;
persistent err_A2;
persistent out_A1;
persistent out_A2;

persistent err_C1;
persistent err_C2;
persistent out_C1;
persistent out_C2;

%%对三相静态变量初始化
if isempty(err_A1)
    err_A1 = 0;
end
if isempty(err_A2)
    err_A2 = 0;
end
if isempty(out_A1)
    out_A1 = 0;
end
if isempty(out_A2)
    out_A2 = 0;
end


if isempty(err_C1)
    err_C1 = 0;
end
if isempty(err_C2)
    err_C2 = 0;
end
if isempty(out_C1)
    out_C1 = 0;
end
if isempty(out_C2)
    out_C2 = 0;
end

%%Discrete
t1 = Wc * Ts;
t2 = W0^2 * Ts^2;
t3 = t2 + 4*t1 + 4;

b0 = (Kp*t2 + 4*(Kp+Kr)*t1 + 4*Kp) / t3;
b1 = (2*Kp*t2 - 8*Kp) / t3;
b2 = (Kp*t2 + 4*Kp - 4*(Kp+Kr)*t1) / t3;
a1 = (2*t2 - 8) / t3;
a2 = (t2 - 4*t1 + 4) / t3;
%%限制输出
if b0>3000
    b0=0;
end
if b0<-3000
    b0=0;
end

%%计算三相输出量
out_A = b0*err_A + b1*err_A1 + b2*err_A2 - a1*out_A1 - a2*out_A2;
out_A2 = out_A1;
out_A1 = out_A;
err_A2 = err_A1;
err_A1 = err_A;


out_C = b0*err_C + b1*err_C1 + b2*err_C2 - a1*out_C1 - a2*out_C2;
out_C2 = out_C1;
out_C1 = out_C;
err_C2 = err_C1;
err_C1 = err_C;

== matlab function Dual_Three_Leg_Inverter_DPWMA/Digital PR ABC/Discrete QPR 3ph ==
  settings: updateMethod=DISCRETE  sampleTime=Ts
  data: err_A input; err_B input; err_C input; out_A output; Kp input; Kr input; Wc input; Ts input; out_B output; out_C output
function [out_A, out_B, out_C] = fcn(err_A, err_B, err_C, Kp, Kr, Wc, Ts)

W0 = 50*2*pi;

%%定义三相静态变量
persistent err_A1;
persistent err_A2;
persistent out_A1;
persistent out_A2;

persistent err_B1;
persistent err_B2;
persistent out_B1;
persistent out_B2;

persistent err_C1;
persistent err_C2;
persistent out_C1;
persistent out_C2;

%%对三相静态变量初始化
if isempty(err_A1)
    err_A1 = 0;
end
if isempty(err_A2)
    err_A2 = 0;
end
if isempty(out_A1)
    out_A1 = 0;
end
if isempty(out_A2)
    out_A2 = 0;
end

if isempty(err_B1)
    err_B1 = 0;
end
if isempty(err_B2)
    err_B2 = 0;
end
if isempty(out_B1)
    out_B1 = 0;
end
if isempty(out_B2)
    out_B2 = 0;
end

if isempty(err_C1)
    err_C1 = 0;
end
if isempty(err_C2)
    err_C2 = 0;
end
if isempty(out_C1)
    out_C1 = 0;
end
if isempty(out_C2)
    out_C2 = 0;
end

%%Discrete
t1 = Wc * Ts;
t2 = W0^2 * Ts^2;
t3 = t2 + 4*t1 + 4;

b0 = (Kp*t2 + 4*(Kp+Kr)*t1 + 4*Kp) / t3;
b1 = (2*Kp*t2 - 8*Kp) / t3;
b2 = (Kp*t2 + 4*Kp - 4*(Kp+Kr)*t1) / t3;
a1 = (2*t2 - 8) / t3;
a2 = (t2 - 4*t1 + 4) / t3;

%%计算三相输出量
out_A = b0*err_A + b1*err_A1 + b2*err_A2 - a1*out_A1 - a2*out_A2;
out_A2 = out_A1;
out_A1 = out_A;
err_A2 = err_A1;
err_A1 = err_A;

out_B = b0*err_B + b1*err_B1 + b2*err_B2 - a1*out_B1 - a2*out_B2;
out_B2 = out_B1;
out_B1 = out_B;
err_B2 = err_B1;
err_B1 = err_B;

out_C = b0*err_C + b1*err_C1 + b2*err_C2 - a1*out_C1 - a2*out_C2;
out_C2 = out_C1;
out_C1 = out_C;
err_C2 = err_C1;
err_C1 = err_C;
